simulink model "inversor"  (R2026b)
settings: Solver=VariableStepAuto  StopTime=40  MaxStep=1e-3
InitFcn:
  | run("C:\Users\ArnauCoronado\Documents_local\master\gedit\practica_ppc_Arnau_Coronado_Nadal_gedit\simulacio_2\inversor_param.m")
values from neighbouring files (symbols this model uses):
  P_disp = [500 500 2000 2000 2000]    [inversor_param.m]
  P_init = min(alpha_0*Pn_inv, P_disp)    [inversor_param.m]
  Pn_inv = 2000    [inversor_param.m]
  rate_transition_init_val = alpha_0    (= 0.5)    [inversor_param.m]
  sample_time = 0.2    [inversor_param.m]
  step_time = 10    [inversor_param.m]
  step_time2 = 20    [inversor_param.m]
  t_delay_com = 20e-3    (= 0.02)    [inversor_param.m]
  tau_pv = 0.5    [inversor_param.m]
  transp_delay_init_outp = alpha_0    (= 0.5)    [inversor_param.m]
  transp_delay_pppc_meas = Pppc_0    [inversor_param.m]
libraries: sl_discontinuities x5
settings Model: Creator=arnau.coronado  LastModifiedBy=ArnauCoronado

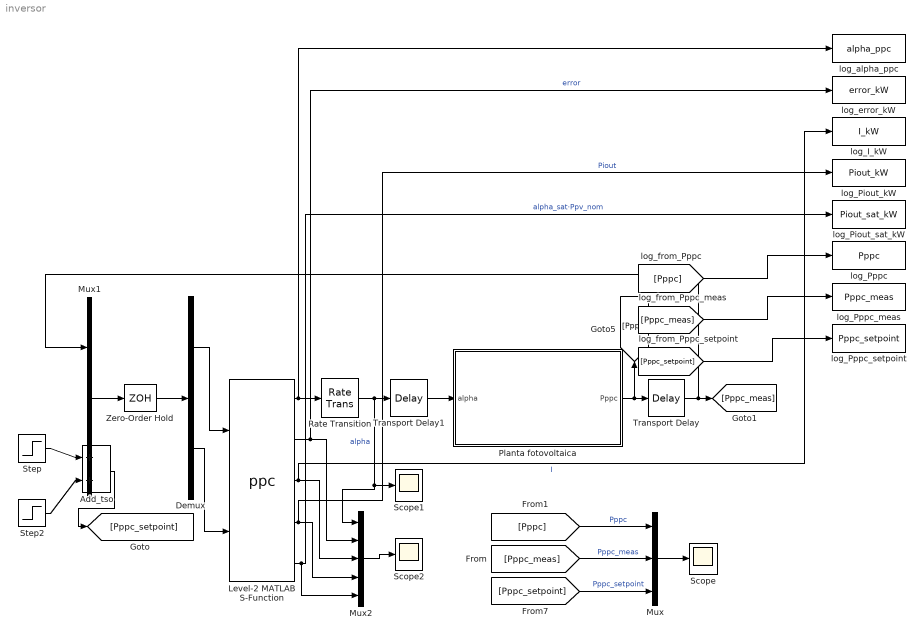
== system inversor ==
  Add_tso : Sum
  Demux : Demux  Outputs=2
  Level-2 MATLAB S-Function : M-S-Function  FunctionName=ppc  Parameters=sample_time, Ppv_nom, Ki, Kp, Ramp_rate_lim, ppc_init_value, antiwindup
  Mux : Mux  Inputs=3
  Mux1 : Mux  Inputs=2
  Mux2 : Mux  Inputs=5
  Planta fotovoltaica : Subsystem
  Rate Transition : RateTransition  InitialCondition=rate_transition_init_val
  Scope : Scope
      settings: ActiveDisplayYMinimum=-1249.9999999999998  ActiveDisplayYMaximum=11250  YLabel=Power [kW]
  Scope1 : Scope
      settings: ActiveDisplayYMinimum=0.51151891137932926  ActiveDisplayYMaximum=1.0542756765134078  YLabel=Power [kW]  DataLoggingVariableName=ScopeData2
  Scope2 : Scope
      settings: ActiveDisplayYMinimum=-3229.6576004897333  ActiveDisplayYMaximum=8136.6286222766366  YLabel=Power [kW]  DataLoggingVariableName=ScopeData3
  Step : Step  Time=step_time  InitialValue=P_tso_ini  FinalValue=P_tso_fin  SampleTime=0
  Step2 : Step  Time=step_time2  FinalValue=P_tso_delta2  SampleTime=0
  Transport Delay : TransportDelay  DelayTime=t_delay_com  InitialOutput=transp_delay_pppc_meas
  Transport Delay1 : TransportDelay  DelayTime=t_delay_com  InitialOutput=transp_delay_init_outp
  Zero-Order Hold : ZeroOrderHold  SampleTime=sample_time
  log_I_kW : ToWorkspace  VariableName=I_kW  SaveFormat=Timeseries  SampleTime=0.01
  log_Piout_kW : ToWorkspace  VariableName=Piout_kW  SaveFormat=Timeseries  SampleTime=0.01
  log_Piout_sat_kW : ToWorkspace  VariableName=Piout_sat_kW  SaveFormat=Timeseries  SampleTime=0.01
  log_Pppc : ToWorkspace  VariableName=Pppc  SaveFormat=Timeseries  SampleTime=0.01
  log_Pppc_meas : ToWorkspace  VariableName=Pppc_meas  SaveFormat=Timeseries  SampleTime=0.01
  log_Pppc_setpoint : ToWorkspace  VariableName=Pppc_setpoint  SaveFormat=Timeseries  SampleTime=0.01
  log_alpha_ppc : ToWorkspace  VariableName=alpha_ppc  SaveFormat=Timeseries  SampleTime=0.01
  log_error_kW : ToWorkspace  VariableName=error_kW  SaveFormat=Timeseries  SampleTime=0.01
  wires:
  Mux/1 -> Scope/1
  [Pppc_meas] -> Mux/2  "Pppc_meas"
  Transport Delay/1 -> Mux1/1, [Pppc_meas]
  Mux1/1 -> Zero-Order Hold/1
  Zero-Order Hold/1 -> Demux/1
  Demux/1 -> Level-2 MATLAB S-Function/1
  Demux/2 -> Level-2 MATLAB S-Function/2
  Planta fotovoltaica/1(Pppc) -> Transport Delay/1, [Pppc]
  Level-2 MATLAB S-Function/1 -> Rate Transition/1, log_alpha_ppc/1
  Rate Transition/1 -> Mux2/1, Scope1/1, Transport Delay1/1  "alpha"
  [Pppc_setpoint] -> Mux/3  "Pppc_setpoint"
  [Pppc] -> Mux/1  "Pppc"
  Transport Delay1/1 -> Planta fotovoltaica/1(alpha)
  Mux2/1 -> Scope2/1
  Level-2 MATLAB S-Function/5 -> Mux2/5, log_Piout_sat_kW/1  "alpha_sat·Ppv_nom"
  Level-2 MATLAB S-Function/4 -> Mux2/4, log_Piout_kW/1  "Piout"
  Level-2 MATLAB S-Function/3 -> Mux2/3, log_I_kW/1  "I"
  Level-2 MATLAB S-Function/2 -> Mux2/2, log_error_kW/1  "error"
  [Pppc] -> log_Pppc/1
  [Pppc_meas] -> log_Pppc_meas/1
  [Pppc_setpoint] -> log_Pppc_setpoint/1
  Step/1 -> Add_tso/1
  Step2/1 -> Add_tso/2
  Add_tso/1 -> [Pppc_setpoint]

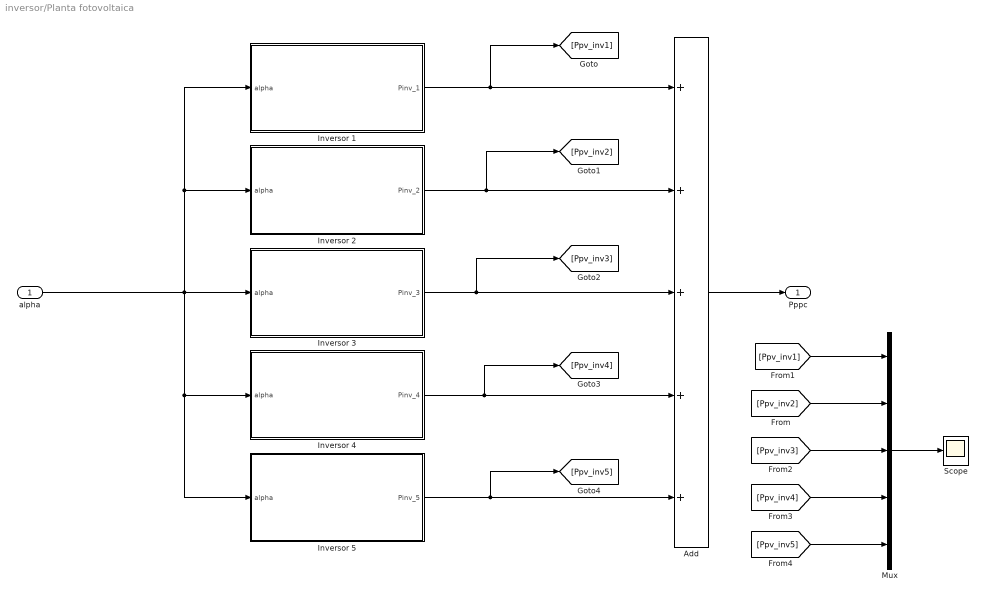
== system inversor/Planta fotovoltaica ==
  alpha : Inport
  Add : Sum  Inputs=+++++
  Inversor 1 : Subsystem
  Inversor 2 : Subsystem
  Inversor 3 : Subsystem
  Inversor 4 : Subsystem
  Inversor 5 : Subsystem
  Mux : Mux  Inputs=5
  Scope : Scope
      settings: ActiveDisplayYMinimum=-264.44761279829225  ActiveDisplayYMaximum=2491.8023717590063
  Pppc : Outport
  wires:
  Inversor 3/1(Pinv_3) -> Add/3, [Ppv_inv3]
  Inversor 2/1(Pinv_2) -> [Ppv_inv2], Add/2
  Inversor 5/1(Pinv_5) -> Add/5, [Ppv_inv5]
  Inversor 4/1(Pinv_4) -> [Ppv_inv4], Add/4
  Inversor 1/1(Pinv_1) -> Add/1, [Ppv_inv1]
  alpha/1 -> Inversor 4/1(alpha), Inversor 5/1(alpha), Inversor 3/1(alpha), Inversor 2/1(alpha), Inversor 1/1(alpha)
  Add/1 -> Pppc/1
  [Ppv_inv5] -> Mux/5
  [Ppv_inv4] -> Mux/4
  Mux/1 -> Scope/1
  [Ppv_inv3] -> Mux/3
  [Ppv_inv2] -> Mux/2
  [Ppv_inv1] -> Mux/1

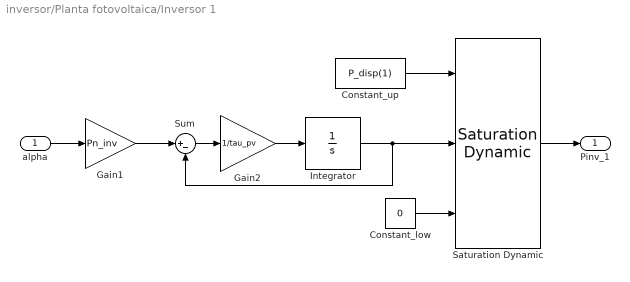
== system inversor/Planta fotovoltaica/Inversor 1 ==
  alpha : Inport
  Constant_low : Constant  Value=0
  Constant_up : Constant  Value=P_disp(1)
  Gain1 : Gain  Gain=Pn_inv
  Gain2 : Gain  Gain=1/tau_pv
  Integrator : Integrator  InitialCondition=P_init(1)
  Saturation Dynamic : sl_discontinuities/Saturation Dynamic  OutMin=[]  OutMax=[]  OutDataTypeStr=Inherit: Same as second input  OutDataType=fixdt(1, 16)  OutScaling=2^-10  DoSatur=off
      settings: LibrarySourceBlock=|
      | simulink/Discontinuities/Saturation
      | Dynamic
  Sum : Sum  Inputs=|+-
  Pinv_1 : Outport
  wires:
  alpha/1 -> Gain1/1
  Integrator/1 -> Sum/2, Saturation Dynamic/2
  Saturation Dynamic/1 -> Pinv_1/1
  Gain1/1 -> Sum/1
  Sum/1 -> Gain2/1
  Constant_low/1 -> Saturation Dynamic/3
  Gain2/1 -> Integrator/1
  Constant_up/1 -> Saturation Dynamic/1

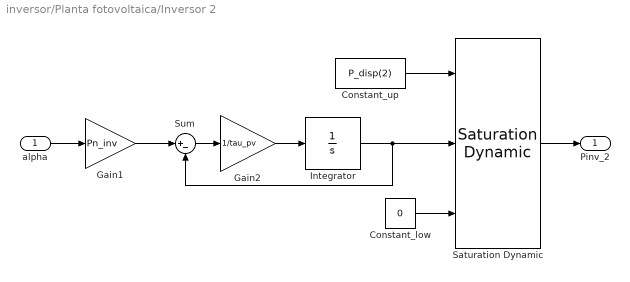
== system inversor/Planta fotovoltaica/Inversor 2 ==
  alpha : Inport
  Constant_low : Constant  Value=0
  Constant_up : Constant  Value=P_disp(2)
  Gain1 : Gain  Gain=Pn_inv
  Gain2 : Gain  Gain=1/tau_pv
  Integrator : Integrator  InitialCondition=P_init(2)
  Saturation Dynamic : sl_discontinuities/Saturation Dynamic  OutMin=[]  OutMax=[]  OutDataTypeStr=Inherit: Same as second input  OutDataType=fixdt(1, 16)  OutScaling=2^-10  DoSatur=off
      settings: LibrarySourceBlock=|
      | simulink/Discontinuities/Saturation
      | Dynamic
  Sum : Sum  Inputs=|+-
  Pinv_2 : Outport
  wires:
  Constant_up/1 -> Saturation Dynamic/1
  Gain2/1 -> Integrator/1
  Constant_low/1 -> Saturation Dynamic/3
  Sum/1 -> Gain2/1
  Gain1/1 -> Sum/1
  Saturation Dynamic/1 -> Pinv_2/1
  Integrator/1 -> Saturation Dynamic/2, Sum/2
  alpha/1 -> Gain1/1

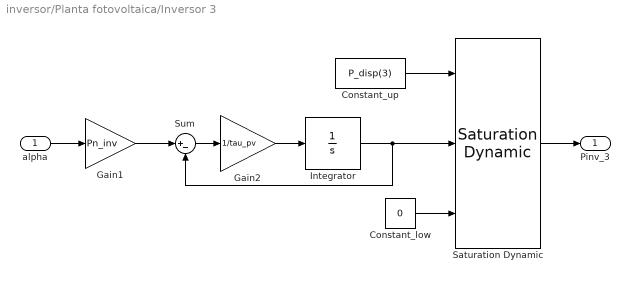
== system inversor/Planta fotovoltaica/Inversor 3 ==
  alpha : Inport
  Constant_low : Constant  Value=0
  Constant_up : Constant  Value=P_disp(3)
  Gain1 : Gain  Gain=Pn_inv
  Gain2 : Gain  Gain=1/tau_pv
  Integrator : Integrator  InitialCondition=P_init(3)
  Saturation Dynamic : sl_discontinuities/Saturation Dynamic  OutMin=[]  OutMax=[]  OutDataTypeStr=Inherit: Same as second input  OutDataType=fixdt(1, 16)  OutScaling=2^-10  DoSatur=off
      settings: LibrarySourceBlock=|
      | simulink/Discontinuities/Saturation
      | Dynamic
  Sum : Sum  Inputs=|+-
  Pinv_3 : Outport
  wires:
  alpha/1 -> Gain1/1
  Integrator/1 -> Sum/2, Saturation Dynamic/2
  Saturation Dynamic/1 -> Pinv_3/1
  Gain1/1 -> Sum/1
  Sum/1 -> Gain2/1
  Constant_low/1 -> Saturation Dynamic/3
  Gain2/1 -> Integrator/1
  Constant_up/1 -> Saturation Dynamic/1

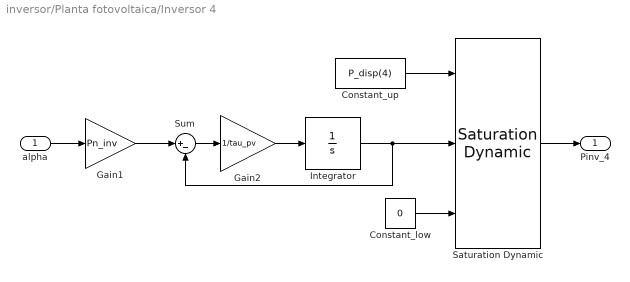
== system inversor/Planta fotovoltaica/Inversor 4 ==
  alpha : Inport
  Constant_low : Constant  Value=0
  Constant_up : Constant  Value=P_disp(4)
  Gain1 : Gain  Gain=Pn_inv
  Gain2 : Gain  Gain=1/tau_pv
  Integrator : Integrator  InitialCondition=P_init(4)
  Saturation Dynamic : sl_discontinuities/Saturation Dynamic  OutMin=[]  OutMax=[]  OutDataTypeStr=Inherit: Same as second input  OutDataType=fixdt(1, 16)  OutScaling=2^-10  DoSatur=off
      settings: LibrarySourceBlock=|
      | simulink/Discontinuities/Saturation
      | Dynamic
  Sum : Sum  Inputs=|+-
  Pinv_4 : Outport
  wires:
  Constant_up/1 -> Saturation Dynamic/1
  Gain2/1 -> Integrator/1
  Constant_low/1 -> Saturation Dynamic/3
  Sum/1 -> Gain2/1
  Gain1/1 -> Sum/1
  Saturation Dynamic/1 -> Pinv_4/1
  Integrator/1 -> Saturation Dynamic/2, Sum/2
  alpha/1 -> Gain1/1

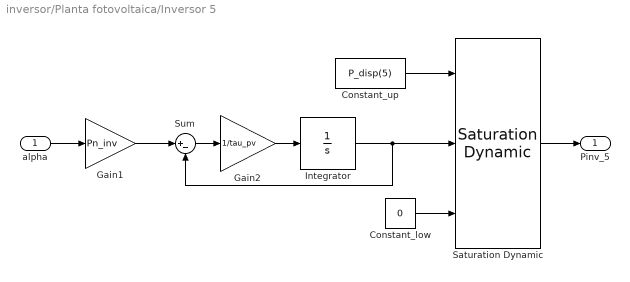
== system inversor/Planta fotovoltaica/Inversor 5 ==
  alpha : Inport
  Constant_low : Constant  Value=0
  Constant_up : Constant  Value=P_disp(5)
  Gain1 : Gain  Gain=Pn_inv
  Gain2 : Gain  Gain=1/tau_pv
  Integrator : Integrator  InitialCondition=P_init(5)
  Saturation Dynamic : sl_discontinuities/Saturation Dynamic  OutMin=[]  OutMax=[]  OutDataTypeStr=Inherit: Same as second input  OutDataType=fixdt(1, 16)  OutScaling=2^-10  DoSatur=off
      settings: LibrarySourceBlock=|
      | simulink/Discontinuities/Saturation
      | Dynamic
  Sum : Sum  Inputs=|+-
  Pinv_5 : Outport
  wires:
  alpha/1 -> Gain1/1
  Integrator/1 -> Sum/2, Saturation Dynamic/2
  Saturation Dynamic/1 -> Pinv_5/1
  Gain1/1 -> Sum/1
  Sum/1 -> Gain2/1
  Constant_low/1 -> Saturation Dynamic/3
  Gain2/1 -> Integrator/1
  Constant_up/1 -> Saturation Dynamic/1
